simulink model "Exp_3_P_O"  (R2025a)
settings: Solver=ode23tb  StartTime=0.0  StopTime=1  RelTol=1e-3
libraries: spsSeriesRLCBranchLib x4, spsCurrentMeasurementLib x1, spsDiodeLib x1, spsIGBTLib x1, spsPVArrayLib x1, spsPWMGeneratorDCDCLib x1, spsVoltageMeasurementLib x1, sps_lib x1
settings Model: Creator=ASUS  LastModifiedBy=ASUS

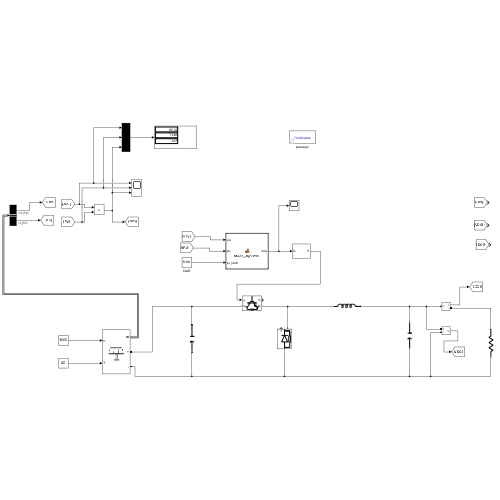
[thumbnail: Simulink's stored preview of the top-level diagram]
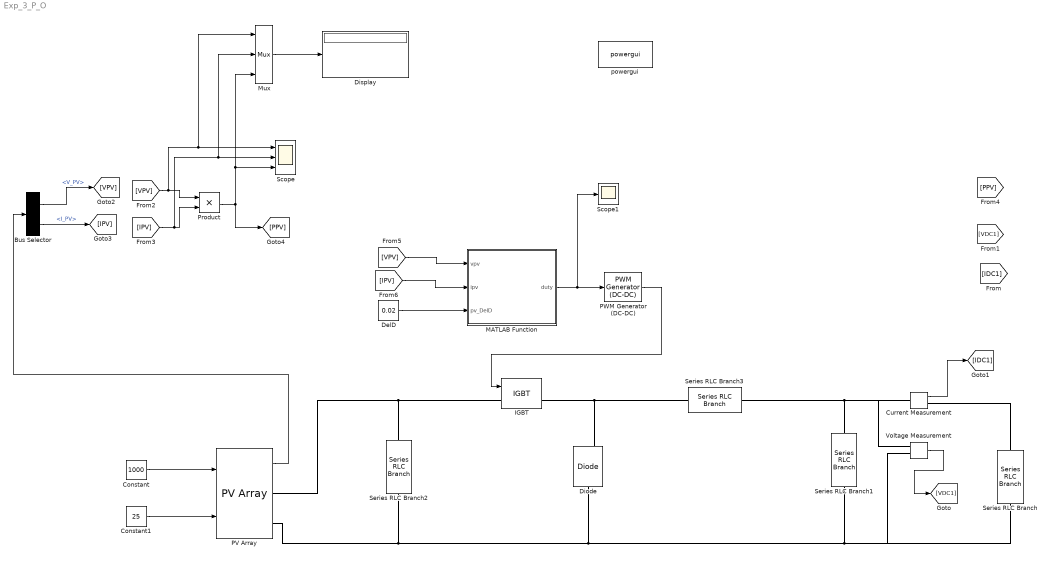
== system Exp_3_P_O ==
  Bus Selector : BusSelector  OutputSignals=V_PV,I_PV
  Constant : Constant  Value=1000
  Constant1 : Constant  Value=25
  Current Measurement : spsCurrentMeasurementLib/Current Measurement  PhasorSimulation=off  OutputType=Complex  PSBequivalent=0
  DelD : Constant  Value=0.02
  Diode : spsDiodeLib/Diode  Ron=0.001  Lon=0  Vf=0.8  IC=0  UseSnubber=0  Rs=500  Cs=250e-9  Measurements=on
  Display : Display
  IGBT : spsIGBTLib/IGBT  Ron=0.001  Lon=0  Vf=1  Tf=1e-6  Tt=2e-6  IC=0  Rs=1e5  Cs=inf  Measurements=on
  MATLAB Function : MATLAB Function  TreatAsAtomicUnit=on
  Mux : Mux  Inputs=3
  PV Array : spsPVArrayLib/PV Array  Npar=1  Nser=3  PlotType=array @ 1000 W/m2 & specified temperatures  S_vec="[ 1000  500  100 ]"  Temp_C_vec="[ 45 25  ]"  ModuleName=User-defined  PlotWhenSelected=off  Pm=213.15  Ncell=60  Voc=36.3  Isc=7.84  Vm=29  Im=7.35  beta_Voc_pc=-0.36099  alpha_Isc_pc=0.102  beta_Voc=-0.13104  alpha_Isc=0.0079968  IL=7.8654  I0=2.9273e-10  nI=0.98119  Rsh=313.0553  Rs=0.39381  RobustModel=off  RobustCellTemperature=313.3991  BAL=on  Tc=1e-6  Tfilter=5e-5
  PWM Generator (DC-DC) : spsPWMGeneratorDCDCLib/PWM Generator (DC-DC)  Fsw=5000  Ts=0
  Product : Product
  Scope : Scope  NumInputPorts=3
      settings: ActiveDisplayYMinimum=-11.822025698744946  ActiveDisplayYMaximum=106.39823128870454
  Scope1 : Scope
      settings: ActiveDisplayYMinimum=0.47000000000000003  ActiveDisplayYMaximum=0.57000000000000017
  Series RLC Branch : spsSeriesRLCBranchLib/Series RLC Branch  LConnTagsString=__new0  RConnTagsString=__new0  BranchType=R  Resistance=3.5  Inductance=1e-3  SetiL0=off  InitialCurrent=0  Capacitance=1e-6  Setx0=off  InitialVoltage=0  Measurements=None
  Series RLC Branch1 : spsSeriesRLCBranchLib/Series RLC Branch  LConnTagsString=__new0  RConnTagsString=__new0  BranchType=C  Resistance=10  Inductance=1e-3  SetiL0=off  InitialCurrent=0  Capacitance=1000e-6  Setx0=off  InitialVoltage=0  Measurements=None
  Series RLC Branch2 : spsSeriesRLCBranchLib/Series RLC Branch  LConnTagsString=__new0  RConnTagsString=__new0  BranchType=C  Resistance=10  Inductance=1e-3  SetiL0=off  InitialCurrent=0  Capacitance=1000e-6  Setx0=off  InitialVoltage=0  Measurements=None
  Series RLC Branch3 : spsSeriesRLCBranchLib/Series RLC Branch  LConnTagsString=__new0  RConnTagsString=__new0  BranchType=L  Resistance=10  Inductance=1e-3  SetiL0=off  InitialCurrent=0  Capacitance=1000e-6  Setx0=off  InitialVoltage=0  Measurements=None
  Voltage Measurement : spsVoltageMeasurementLib/Voltage Measurement  PhasorSimulation=off  OutputType=Complex  PSBequivalent=0
  powergui : sps_lib/powergui  Priority=1  SimulationMode=Continuous  SampleTime=50e-6  frequency=60  Iterations=50  frequencyindice=0  Pbase=100e6  ErrMax=1e-4  UnitsV=kV  UnitsW=MW  buscounter=0  FunctionMessages=off  echomessages=off  EnableUseOfTLC=off  CurrentSourceSwitches=off  DisableSnubberDevices=off  DisableRonSwitches=off  DisableVfSwitches=off  DisplayEquations=off  AutomaticDiscreteSolvers=off  SolverType=Tustin/Backward Euler (TBE)  Interpol=off  ExternalGateDelay=off  methode=off  Ts=100  x0status=blocks  SPID=on  SwTol=0  HookPort=off  NonlinearTolerance=1e-4  nMaxIteration=100  ContinueOnMaxIteration=off  RestoreLinks=warning  ResistiveCurrentMeasurement=off  Frange=[0:2:500]  Ylog=off  Xlog=on  ShowGrid=off  save=off  variable=ZData  structure=0  ZoomFFT=off  StartTime=0.0  cycles=1  DisplayStyle=1  fundamental=60  FreqAxis=off  MaxFrequency=1000  frequencyindicesteady=1  RmsSteady=1  display=off
  wires:
  Constant1/1 -> PV Array/2
  Constant/1 -> PV Array/1
  Voltage Measurement/1 -> [VDC1]
  Current Measurement/1 -> [IDC1]
  PV Array/1 -> Bus Selector/1
  [IPV] -> Mux/2, Scope/2, Product/2
  [VPV] -> Mux/1, Scope/1, Product/1
  Product/1 -> [PPV], Mux/3, Scope/3
  Mux/1 -> Display/1
  PWM Generator (DC-DC)/1 -> IGBT/1
  MATLAB Function/1(duty) -> Scope1/1, PWM Generator (DC-DC)/1
  DelD/1 -> MATLAB Function/3(pv_DelD)
  [VPV] -> MATLAB Function/1(vpv)
  [IPV] -> MATLAB Function/2(ipv)
  Bus Selector/1 -> [VPV]  "<V_PV>"
  Bus Selector/2 -> [IPV]  "<I_PV>"
  connections:
  IGBT/RConn1 -- Diode/RConn1 -- Series RLC Branch3/RConn1
  IGBT/LConn1 -- Series RLC Branch2/LConn1 -- PV Array/RConn1
  Series RLC Branch3/LConn1 -- Voltage Measurement/LConn1 -- Current Measurement/LConn1 -- Series RLC Branch1/LConn1
  Series RLC Branch2/RConn1 -- PV Array/RConn2 -- Voltage Measurement/LConn2 -- Series RLC Branch/RConn1 -- Series RLC Branch1/RConn1 -- Diode/LConn1
  Series RLC Branch/LConn1 -- Current Measurement/RConn1

== matlab function Exp_3_P_O/MATLAB Function ==
  settings: updateMethod=DISCRETE  sampleTime=0.02
  data: vpv input; duty output; ipv input; pv_DelD input
function duty = MPPT_Algorithm(vpv, ipv, pv_DelD)
duty_init=0.5;
duty_min=0;
duty_max=0.85;
delta=pv_DelD;
persistent Vold Pold duty_old;
if isempty(Vold)
    Vold=0;
    Pold=0;
    duty_old=duty_init;
end
P=vpv*ipv;
dv=vpv-Vold;
dp=P-Pold;
if dp~=0 && vpv>1
    if dp<0
        if dv<0
            duty=duty_old-delta;
        else
            duty=duty_old+delta;
        end
    else
        if dv<0
            duty=duty_old+delta;
        else
            duty=duty_old-delta;

        end
    end
else
    duty=duty_old;
end
if duty>=duty_max
    duty=duty_max;
elseif duty<duty_min
    duty=duty_min;
end
duty_old=duty;
Vold=vpv;
Pold=P;
